simulink model "Buck_MPC"  (R2023b)
settings: Solver=VariableStepAuto  StartTime=0.0  StopTime=0.1  FixedStep=1e-6  RelTol=1e-3
libraries: spsSeriesRLCBranchLib x5, spsVoltageMeasurementLib x3, spsCurrentMeasurementLib x2, simulink x2, spsMosfetLib x2, spsDCVoltageSourceLib x1, spsControlledCurrentSourceLib x1, slpidlib x1, sps_lib x1
settings Model: SimulationMode=accelerator  Creator=45276  LastModifiedBy=45276

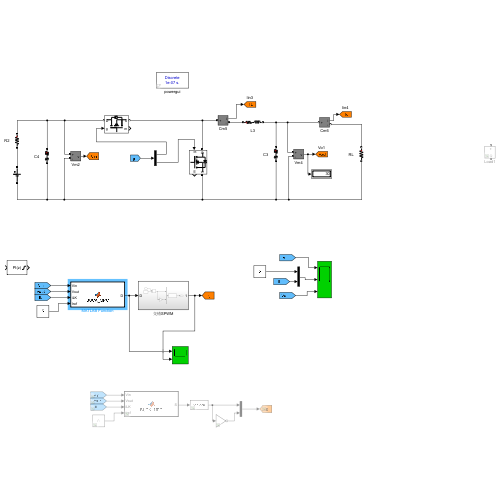
[thumbnail: Simulink's stored preview of the top-level diagram]
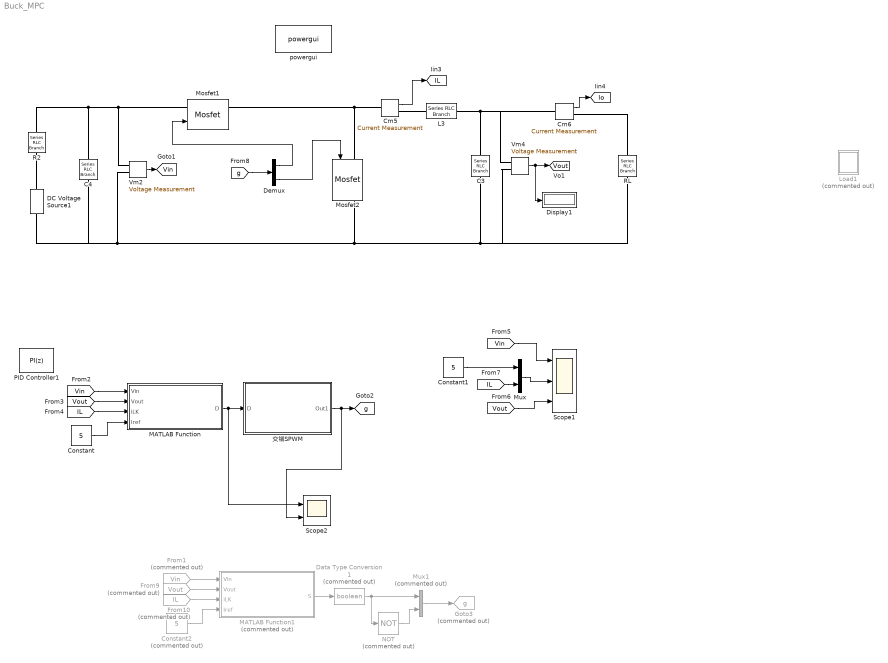
== system Buck_MPC ==
  C3 : spsSeriesRLCBranchLib/Series RLC Branch  LConnTagsString=__new0  RConnTagsString=__new0  BranchType=RC  Resistance=0.015  Inductance=0  SetiL0=off  InitialCurrent=0  Capacitance=100e-6  Setx0=on  InitialVoltage=20  Measurements=None
  C4 : spsSeriesRLCBranchLib/Series RLC Branch  LConnTagsString=__new0  RConnTagsString=__new0  BranchType=RC  Resistance=0.01  Inductance=0  SetiL0=off  InitialCurrent=0  Capacitance=1e-6  Setx0=on  InitialVoltage=24  Measurements=None
  Cm5 : spsCurrentMeasurementLib/Current Measurement  PhasorSimulation=off  OutputType=Complex  PSBequivalent=0
  Cm6 : spsCurrentMeasurementLib/Current Measurement  PhasorSimulation=off  OutputType=Complex  PSBequivalent=0
  Constant : Constant  Value=5
  Constant1 : Constant  Value=5
  Constant2 : Constant  Commented=on  Value=5
  DC Voltage Source1 : spsDCVoltageSourceLib/DC Voltage Source  Amplitude=60  Measurements=None
  Data Type Conversion1 : DataTypeConversion  Commented=on  OutDataTypeStr=boolean  SaturateOnIntegerOverflow=off  RndMeth=Floor
  Demux : Demux  Outputs=2
  Display1 : Display
  From1 : From  Commented=on  GotoTag=Vin  TagVisibility=global
      settings: CloseFcn=tagdialog Close
  From10 : From  Commented=on  GotoTag=IL  TagVisibility=global
      settings: CloseFcn=tagdialog Close
  From9 : From  Commented=on  GotoTag=Vout  TagVisibility=global
      settings: CloseFcn=tagdialog Close
  Goto3 : Goto  Commented=on  GotoTag=g  TagVisibility=global
  L3 : spsSeriesRLCBranchLib/Series RLC Branch  LConnTagsString=__new0  RConnTagsString=__new0  BranchType=RL  Resistance=0.2  Inductance=10e-4  SetiL0=off  InitialCurrent=0  Capacitance=inf  Setx0=off  InitialVoltage=0  Measurements=None
  Load1 : Subsystem  Commented=on  mask{Vst1=[3 3 8 8 5 5 2 2].', Tst1=[0 0.01 0.01+eps 0.02 0.02+eps 0.025 0.025+eps 0.03].', Tstsp=1e-8}
      mask prompts: Vst1 "突变值Vst1, eg:[3 3 8 8 2 2].'"; Tst1 "突变时间Tst1, eg:[0 0.01 0.01+eps 0.02 0.02+eps 0.03].'"; Tstsp "采样时间Tstsp"
      settings: PortSchema="{\"entries\":[{\"content\":{\"sides\":[{\"content\":{},\"type\":\"ConnectorPlacement.EquallySpacedRectSide\",\"uuid\":\"4352356a-a73d-4efd-aeba-c61bfc863045\"},{\"content\":{\"side\":\"RIGHT\"},\"type\":\"ConnectorPlacement.EquallySpacedRectSide\",\"uuid\":\"a043c14f-179e-462d-8cc8-5b83a7edcd21\"},{\"content\":{\"connectorIds\":[\"LConn1\"],\"side\":\"TOP\"},\"type\":\"ConnectorPlacement.EquallySpacedRectSide\",\"uuid\":\"f8810edc-586f-49c6-95ea-bd3a7aa2b56d\"},{\"content\":{\"connectorIds\":[\"RConn1\"],\"side\":\"BOTTOM\"},\"type\":\"ConnectorPlacement.EquallySpacedRectSide\",\"uuid\":\"956d2570-7b82-4c39-8513-d9bfab6f6be6\"}]},\"type\":\"ConnectorPlacement.EquallySpacedConnector\",\"uuid\":\"2f028cb1-1f36-487b-8c9b-3c22934b1877\"}],\"packageUris\":[\"http://schema.mathworks.com/mf0/Connector/R2020b\"],\"version\":\"1.0\"}"
      mask DialogControl ParameterGroupVar Prompt: 参数
  MATLAB Function : MATLAB Function  TreatAsAtomicUnit=on
  MATLAB Function1 : MATLAB Function  Commented=on  TreatAsAtomicUnit=on
  Mosfet1 : spsMosfetLib/Mosfet  Ron=0.1  Lon=0  Rd=0.01  Vfd=0  IC=0  Rs=1e5  Cs=inf  Measurements=on
  Mosfet2 : spsMosfetLib/Mosfet  Ron=0.1  Lon=0  Rd=0.01  Vfd=0  IC=0  Rs=1e5  Cs=inf  Measurements=on
  Mux : Mux  Inputs=2
  Mux1 : Mux  Commented=on  Inputs=2
  NOT : Logic  Commented=on  Operator=NOT  IconShape=distinctive  AllPortsSameDT=off  OutDataTypeStr=boolean
  PID Controller1 : slpidlib/PID Controller  Controller=PI  Form=Parallel  TimeDomain=Discrete-time  UseExternalTs=off  SampleTime=-1  IntegratorMethod=Forward Euler  FilterMethod=Forward Euler  ControllerParametersSource=internal  P=1  I=1  UseKiTs=off  D=0  N=100  UseFilter=on  TunerSelectOption=Transfer Function Based (PID Tuner App)  InitialConditionSource=internal  InitialConditionForIntegrator=0  InitialConditionForFilter=0  DifferentiatorICPrevScaledInput=0  ExternalReset=none  TrackingMode=off  Kt=100  LimitOutput=on  SatLimitsSource=internal  UpperSaturationLimit=1  LowerSaturationLimit=0  LinearizeAsGain=off  AntiWindupMode=none  Kb=1  LimitIntegrator=off  UpperIntegratorSaturationLimit=inf  LowerIntegratorSaturationLimit=-inf  POutMin=[]  POutMax=[]  IOutMin=[]  IOutMax=[]  DOutMin=[]  DOutMax=[]  NOutMin=[]  NOutMax=[]  SumOutMin=[]  SumOutMax=[]  SaturationOutMin=[]  SaturationOutMax=[]  PParamMin=[]  PParamMax=[]  IParamMin=[]  IParamMax=[]  DParamMin=[]  DParamMax=[]  NParamMin=[]  NParamMax=[]  KbParamMin=[]  KbParamMax=[]  KtParamMin=[]  KtParamMax=[]  KbOutMin=[]  KbOutMax=[]  KtOutMin=[]  KtOutMax=[]  IntegratorOutMin=[]  IntegratorOutMax=[]  FilterOutMin=[]  FilterOutMax=[]  SumI1OutMin=[]  SumI1OutMax=[]  SumI2OutMin=[]  SumI2OutMax=[]  SumI3OutMin=[]  SumI3OutMax=[]  SumI4OutMin=[]  SumI4OutMax=[]  SumDOutMin=[]  SumDOutMax=[]  DifferentiatorOutMin=[]  DifferentiatorOutMax=[]  FilterDiffOutCoefMin=[]  FilterDiffOutCoefMax=[]  ReciprocalOutMin=[]  ReciprocalOutMax=[]  SumDenOutMin=[]  SumDenOutMax=[]  SumNumOutMin=[]  SumNumOutMax=[]  DivideOutMin=[]  DivideOutMax=[]  UdiffTsProdOutMin=[]  UdiffTsProdOutMax=[]  NTsProdOutMin=[]  NTsProdOutMax=[]  UintegralTsProdOutMin=[]  UintegralTsProdOutMax=[]  UngainTsProdOutMin=[]  UngainTsProdOutMax=[]  ClampingZeroOutDataTypeStr=Inherit: Inherit via back propagation  ClampingZeroOutMin=[]  ClampingZeroOutMax=[]  FilterDenConstantOutDataTypeStr=Inherit: Inherit via back propagation  FilterDenConstantOutMin=[]  FilterDenConstantOutMax=[]  PCopyOutDataTypeStr=Inherit: Inherit via back propagation  PCopyOutMin=[]  PCopyOutMax=[]  NCopyOutDataTypeStr=Inherit: Inherit via back propagation  NCopyOutMin=[]  NCopyOutMax=[]  IntegratorContinuousStateAttributes=''  IntegratorStateMustResolveToSignalObject=off  IntegratorRTWStateStorageClass=Auto  FilterContinuousStateAttributes=''  FilterStateMustResolveToSignalObject=off  FilterRTWStateStorageClass=Auto  ParallelPVariant=InternalParameters  IdealPVariant=Disabled  IVariant=InternalParameters  DVariant=Disabled  IntegratorVariant=Discrete  SatVariant=Enabled  AWVariant=Passthrough  PCopyVariant=Disabled  TRVariant=Disabled  FdbkBlocksVariant=Forward  IdealPFdbkVariant=Disabled  SatFdbkVariant=Disabled  DerivativeFilterVariant=Disabled  NVariant=Disabled  NCopyVariant=Disabled_SignalSpec  FilterICVariant=Disabled  IntegratorICVariant=InternalICs  ExternalResetVariant=Disabled  TRSumVariant=Passthrough  SumFdbkVariant=Disabled  SumVariant=Sum_PI  TsampFilterVariant=InternalTs  TsampNgainVariant=Passthrough  TsampIntegralVariant=Disabled_SignalSpec  ExternalSaturationOutDataTypeStr=Inherit: Same as second input
  R2 : spsSeriesRLCBranchLib/Series RLC Branch  LConnTagsString=__new0  RConnTagsString=__new0  BranchType=R  Resistance=0.01  Inductance=0  SetiL0=off  InitialCurrent=0  Capacitance=10e-6  Setx0=on  InitialVoltage=24  Measurements=None
  RL : spsSeriesRLCBranchLib/Series RLC Branch  LConnTagsString=__new0  RConnTagsString=__new0  BranchType=R  Resistance=6  Inductance=0  SetiL0=off  InitialCurrent=0  Capacitance=100e-6  Setx0=on  InitialVoltage=20  Measurements=None
  Scope1 : Scope  NumInputPorts=3
  Scope2 : Scope  NumInputPorts=2
  Vm2 : spsVoltageMeasurementLib/Voltage Measurement  PhasorSimulation=off  OutputType=Complex  PSBequivalent=0
  Vm4 : spsVoltageMeasurementLib/Voltage Measurement  PhasorSimulation=off  OutputType=Complex  PSBequivalent=0
  powergui : sps_lib/powergui  Priority=1  SimulationMode=Discrete  SampleTime=1e-7  frequency=60  Iterations=50  frequencyindice=0  Pbase=100e6  ErrMax=1e-4  UnitsV=kV  UnitsW=MW  buscounter=0  FunctionMessages=off  echomessages=off  EnableUseOfTLC=off  CurrentSourceSwitches=off  DisableSnubberDevices=off  DisableRonSwitches=off  DisableVfSwitches=off  DisplayEquations=off  AutomaticDiscreteSolvers=off  SolverType=Tustin/Backward Euler (TBE)  Interpol=off  ExternalGateDelay=off  methode=off  Ts=100  x0status=blocks  SPID=on  SwTol=0  HookPort=off  NonlinearTolerance=1e-4  nMaxIteration=100  ContinueOnMaxIteration=off  RestoreLinks=warning  ResistiveCurrentMeasurement=off  Frange=[0:2:500]  Ylog=off  Xlog=on  ShowGrid=off  save=off  variable=ZData  structure=0  ZoomFFT=off  StartTime=0.0  cycles=1  DisplayStyle=1  fundamental=60  FreqAxis=off  MaxFrequency=1000  frequencyindicesteady=1  RmsSteady=1  display=off
  交错SPWM : Subsystem
  tag scope: IL=global, Io=global, Vin=global, Vout=global, g=global
  wires:
  Vm2/1 -> [Vin]
  Cm5/1 -> [IL]
  Cm6/1 -> [Io]
  Vm4/1 -> Display1/1, [Vout]
  [Vin] -> MATLAB Function/1(Vin)
  [Vout] -> MATLAB Function/2(Vout)
  [IL] -> MATLAB Function/3(iLK)
  Constant/1 -> MATLAB Function/4(Iref)
  [Vin] -> Scope1/1
  [IL] -> Mux/2
  Constant1/1 -> Mux/1
  Mux/1 -> Scope1/2
  [Vout] -> Scope1/3
  Demux/1 -> Mosfet1/1
  MATLAB Function/1(D) -> Scope2/1, 交错SPWM/1(D)
  交错SPWM/1(Out1) -> Scope2/2, [g]
  [g] -> Demux/1
  Demux/2 -> Mosfet2/1
  From9/1 -> MATLAB Function1/2(Vout)
  Constant2/1 -> MATLAB Function1/4(Iref)
  From1/1 -> MATLAB Function1/1(Vin)
  From10/1 -> MATLAB Function1/3(iLK)
  Mux1/1 -> Goto3/1
  NOT/1 -> Mux1/2
  Data Type Conversion1/1 -> NOT/1, Mux1/1
  MATLAB Function1/1(S) -> Data Type Conversion1/1
  connections:
  Cm5/LConn1 -- Mosfet2/LConn1 -- Mosfet1/RConn1
  C3/LConn1 -- Vm4/LConn1 -- Cm6/LConn1 -- L3/RConn1
  C3/RConn1 -- Vm4/LConn2 -- RL/RConn1 -- Mosfet2/RConn1 -- C4/RConn1 -- DC Voltage Source1/LConn1 -- Vm2/LConn2
  C4/LConn1 -- R2/LConn1 -- Mosfet1/LConn1 -- Vm2/LConn1
  Cm5/RConn1 -- L3/LConn1
  DC Voltage Source1/RConn1 -- R2/RConn1
  RL/LConn1 -- Cm6/RConn1

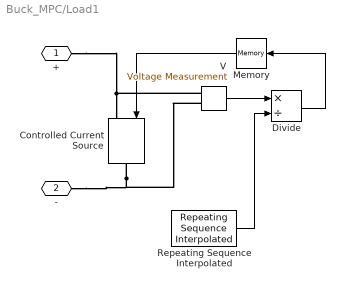
== system Buck_MPC/Load1 ==
  Controlled Current Source : spsControlledCurrentSourceLib/Controlled Current Source  Initialize=on  Source_Type=AC  Amplitude=0  Phase=0  Frequency=0  Measurements=None
  Divide : Product  Inputs=*/
  Memory : Memory
  Repeating Sequence Interpolated : simulink/Sources/Repeating Sequence Interpolated  OutValues=Vst1  TimeValues=Tst1  LookUpMeth=Interpolation-Use End Values  tsamp=Tstsp  OutMin=[]  OutMax=[]  OutDataTypeStr=double  OutputDataTypeScalingMode=double  OutDataType=fixdt(0,8)  OutScaling=2^-10
  V : spsVoltageMeasurementLib/Voltage Measurement  PhasorSimulation=off  OutputType=Complex  PSBequivalent=0
  + : PMIOPort  Side=Left
  - : PMIOPort  Port=2  Side=Right
  wires:
  Memory/1 -> Controlled Current Source/1
  Repeating Sequence Interpolated/1 -> Divide/2
  Divide/1 -> Memory/1
  V/1 -> Divide/1
  connections:
  Controlled Current Source/RConn1 -- -/RConn1 -- V/LConn2
  +/RConn1 -- Controlled Current Source/LConn1 -- V/LConn1

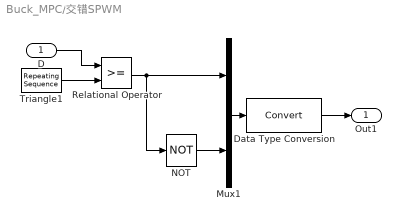
== system Buck_MPC/交错SPWM ==
  D : Inport
  Data Type Conversion : DataTypeConversion  SaturateOnIntegerOverflow=off  RndMeth=Floor
  Mux1 : Mux  Inputs=2
  NOT : Logic  Operator=NOT  IconShape=distinctive  AllPortsSameDT=off  OutDataTypeStr=boolean
  Relational Operator : RelationalOperator  OutDataTypeStr=boolean  InputSameDT=off
  Triangle1 : simulink/Sources/Repeating Sequence  rep_seq_t=[0 1/40000/2 1/40000]  rep_seq_y=[0 1 0]
  Out1 : Outport
  wires:
  Relational Operator/1 -> NOT/1, Mux1/1
  Data Type Conversion/1 -> Out1/1
  Mux1/1 -> Data Type Conversion/1
  Triangle1/1 -> Relational Operator/2
  NOT/1 -> Mux1/2
  D/1 -> Relational Operator/1

== matlab function Buck_MPC/MATLAB Function1 ==
  data: Vin input; S output; Vout input; iLK input; Iref input
function S = BUCK_MPC(Vin, Vout, iLK, Iref)
% 输入定义：
% Vin:  实际采样的输入电压 (V)
% Vout: 实际采样的输出电压 (V)
% iLK:  实际采样的电感电流 (A)
% Iref: 目标电流参考值 (A)

% 1. 模型参数 (必须与电路完全一致)
Ts = 1e-6;      % 采样周期，必须与Simulink求解器步长或触发周期一致
L  = 1e-3;      % 电感 1mH
RL = 0.2;       % 电感内阻

% 2. 初始化代价函数变量
g_opt = 1e10;   % 设为一个很大的初始值，确保第一次比较能成功
S_opt = 0;      % 默认开关状态

% 3. 遍历所有可能的开关状态 (0 和 1)
% State 0: 开关断开 (0V applied to inductor)
% State 1: 开关闭合 (Vin applied to inductor)
possible_states = [0, 1];

for i = 1:2
    u = possible_states(i);
    
    % --- 核心预测模型 (修正点) ---
    % 离散化电感电压方程: L*di/dt = V_sw - Vout - i*R
    % 这里的 V_sw = u * Vin
    % 预测下一时刻电流 i(k+1)
    iLK_next = iLK + (Ts/L) * (u * Vin - Vout - iLK * RL);
    
    % --- 代价函数计算 ---
    % 目标是让预测电流最接近参考电流
    cost = abs(Iref - iLK_next);
    
    % --- 寻优过程 ---
    if cost < g_opt
        g_opt = cost;
        S_opt = u;
    end
end

% 4. 输出最优开关状态
S = S_opt;

== matlab function Buck_MPC/MATLAB Function ==
  data: Vin input; D output; Vout input; iLK input; Iref input
function D = BUCK_MPC(Vin, Vout, iLK, Iref)
% 输出: D (占空比，范围 0-1)

% 1. 参数定义 (必须与电路一致)
Ts = 1/40000;  % 控制周期/PWM周期
L  = 1e-3;      % 电感 1mH
RL = 0.2;       % 电感内阻

% 2. 防止除零错误 (如果Vin还没上电，避免报错)
if Vin < 0.1
    D = 0;
    return;
end

% 3. 无差拍控制核心公式 (Deadbeat Control)
% 反推：为了让 iLK 在 Ts 时间后变为 Iref，需要多大的平均电压？
% 公式拆解：
% delta_I = Iref - iLK;           % 还需要补多少电流
% V_L_req = L * delta_I / Ts;     % 电感两端需要的电压
% V_in_req = V_L_req + Vout + iLK*RL; % 逆推需要的输入侧电压
% D_calc = V_in_req / Vin;        % 归一化为占空比

% 写成一行代码如下：
D_calc = (L * (Iref - iLK) / Ts + Vout + iLK * RL) / Vin;

% 4. 占空比限幅 (Saturation)
% 计算值可能 >1 或 <0，必须限制在物理可行范围内
if D_calc > 0.95        %通常留一点余量，或者直接写 1
    D = 0.95;
elseif D_calc < 0
    D = 0;
else
    D = D_calc;
end
